simulink model "EV_Battery_Discharge_Regen"  (R2023b)
settings: Solver=FixedStepDiscrete  StartTime=0.0  StopTime=1800  FixedStep=.05  RelTol=1e-3
model workspace (MAT data in the model file):
  observer_parameters = [379.525650451 0.0229436828398 29.3915870716 0.534292035398 0.030625 118.171428571 114.285714286 0.1 10]
undefined symbols (not defined in the file or in its folder): Ion, Lithium
libraries: spsControlledCurrentSourceLib x2, spsCurrentMeasurementLib x1, spsGroundLib x1, spsVoltageMeasurementLib x1, spsBatteryLib x1, sps_lib x1
settings Model: Creator=smitp  LastModifiedBy=smitp

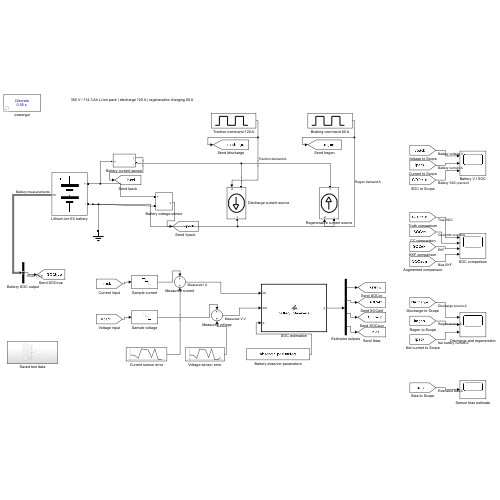
[thumbnail: Simulink's stored preview of the top-level diagram]
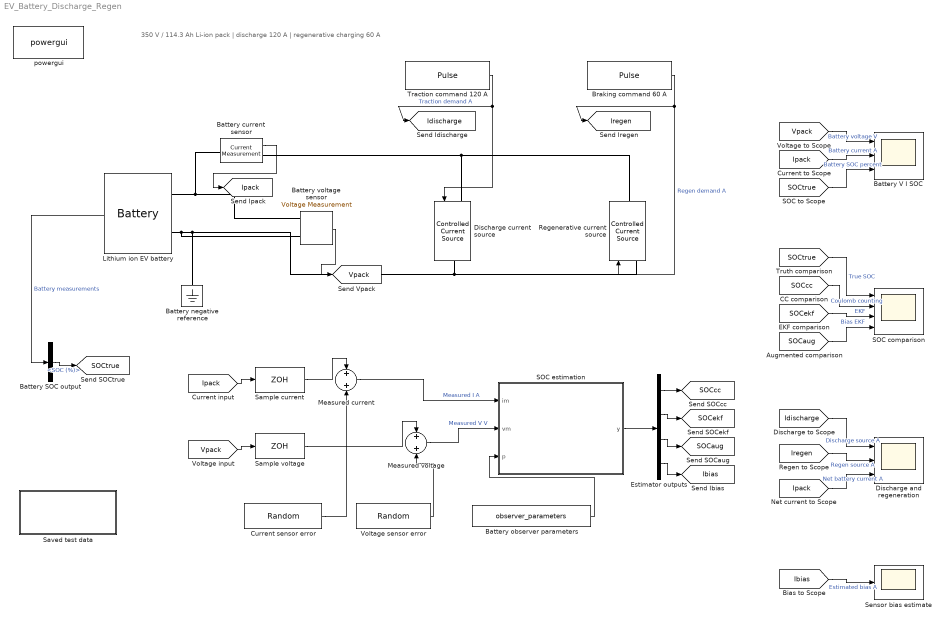
== system EV_Battery_Discharge_Regen ==
  note: 350 V / 114.3 Ah Li-ion pack | discharge 120 A | regenerative charging 60 A
  Battery SOC output : BusSelector  Description=Selects built-in SOC (%) from the Battery measurement bus. It is comparison truth and is never an estimator input.  OutputSignals=SOC (%)
  Battery V I SOC : Scope  NumInputPorts=3
      settings: Description=Primary Scope: voltage, signed battery current and built-in SOC on separate axes.
  Battery current sensor : spsCurrentMeasurementLib/Current Measurement  Description=Measures total battery current. Positive means discharge; negative means charging.  PhasorSimulation=off  OutputType=Complex  PSBequivalent=0
  Battery negative reference : spsGroundLib/Ground  Description=Defines the negative electrical reference node.  LConnTagsString=a
  Battery observer parameters : Constant  Description=Stores E0,K,A,B,R,Qinternal,Qrated,kc,tau extracted from this Battery mask. Contains no true SOC.  Value=observer_parameters
  Battery voltage sensor : spsVoltageMeasurementLib/Voltage Measurement  Description=Connected across the battery terminals to measure pack voltage without drawing current.  PhasorSimulation=off  OutputType=Complex  PSBequivalent=0
  Braking command 60 A : DiscretePulseGenerator  Description=Regeneration is ON from 420 to 540 s in each 600 s cycle, separate from traction.  PulseType=Time based  Amplitude=60  Period=600  PulseWidth=20  PhaseDelay=420
  Current sensor error : RandomNumber  Description=Adds a known +1.2 A offset and 0.25 A standard deviation noise to test current-sensor error.  Mean=1.2  Variance=.25^2  Seed=23  SampleTime=1
  Discharge and regeneration : Scope  NumInputPorts=3
      settings: Description=Shows two nonnegative branch source commands and measured signed net battery current. Ideal-source branch currents equal their commands.
  Discharge current source : spsControlledCurrentSourceLib/Controlled Current Source  Description=Physical current-source load: draws 120 A from HV+ to HV- while traction pulse is high.  Initialize=on  Source_Type=DC  Amplitude=0  Phase=0  Frequency=0  Measurements=None
  Estimator outputs : Demux  Description=Separates the four observer outputs: CC percent, EKF percent, bias-EKF percent, estimated bias A.
  Lithium ion EV battery : spsBatteryLib/Battery  Description=Actual SPS Battery block with internal charge state and nonlinear charge/discharge voltage. This single block represents an EV pack, not a single 350 V cell.  BatType=Lithium-Ion  ShowTempParam=off  ThermalPreset=no  ShowAgeParam=off  NomV=350  NomQ=114.2857142857  SOC=80  Batt_Tr=30  PresetModel=on  MaxQ=114.2857  MinV=262.5  FullV=407.3955  Dis_rate=49.6894  R=0.030625  Normal_OP=103.354  expZone="[378.135      5.614907]"  current=[60 120 180]  Units=Time  Tci=20  NomT=20  T2=-30  MaxQ2=4.8  FullV2=7.1  Normal_OP2=5.655  expZone2="[6.58           1]"  Rca=0.6  ti=2000  Dp=0  Neq0=0  Tsim=1e6  Ta1=25  Qeol=5.4*0.9  Reol=0.013333*1.2  Char_age=[2.3478, 3]  Dis_age=[2.3478, 10]  N1=1500  N2=10500  N3=1000  N4=1400  Ta2=45  N5=950
  Measured current : Sum  Description=Combines true measured current with the current-sensor error.
  Measured voltage : Sum  Description=Combines true terminal voltage with voltage-sensor noise.
  Regenerative current source : spsControlledCurrentSourceLib/Controlled Current Source  Description=Separate physical current source connected in the opposite direction: injects 60 A into the battery positive terminal during braking.  Initialize=on  Source_Type=DC  Amplitude=0  Phase=0  Frequency=0  Measurements=None
  SOC comparison : Scope  NumInputPorts=4
      settings: Description=Shows true SOC, Coulomb counting, EKF and bias-EKF together in percent.
  SOC estimation : MATLAB Function  Description=Online CC, EKF and augmented EKF. States are SOC and filtered current; the augmented filter adds current bias. All priors start at 60 percent.  TreatAsAtomicUnit=on
  Sample current : ZeroOrderHold  Description=Samples measured current once per second for the observer.
  Sample voltage : ZeroOrderHold  Description=Samples terminal voltage at the same 1-second observer rate.
  Saved test data : Subsystem  Description=Records the same Scope signals at 1 s for automated checks and the results table.
  Sensor bias estimate : Scope
      settings: Description=Displays the augmented EKF current-offset estimate. The injected offset is 1.2 A.
  Traction command 120 A : DiscretePulseGenerator  Description=Traction is ON from 60 to 360 s in each 600 s cycle.  PulseType=Time based  Amplitude=120  Period=600  PulseWidth=50  PhaseDelay=60
  Voltage sensor error : RandomNumber  Description=Adds 0.15 V standard deviation pack-voltage noise, with a repeatable independent seed.  Variance=.15^2  Seed=47  SampleTime=1
  powergui : sps_lib/powergui  Description=Solves the connected SPS electrical network. Discrete 50 ms is suitable for this battery current-profile test, not PWM switching.  Priority=1  SimulationMode=Discrete  SampleTime=.05  frequency=60  Iterations=50  frequencyindice=0  Pbase=100e6  ErrMax=1e-4  UnitsV=kV  UnitsW=MW  buscounter=0  FunctionMessages=off  echomessages=off  EnableUseOfTLC=off  CurrentSourceSwitches=off  DisableSnubberDevices=off  DisableRonSwitches=off  DisableVfSwitches=off  DisplayEquations=off  AutomaticDiscreteSolvers=off  SolverType=Tustin/Backward Euler (TBE)  Interpol=off  ExternalGateDelay=off  methode=off  Ts=100  x0status=blocks  SPID=on  SwTol=0  HookPort=off  NonlinearTolerance=1e-4  nMaxIteration=100  ContinueOnMaxIteration=off  RestoreLinks=warning  ResistiveCurrentMeasurement=off  Frange=[0:2:500]  Ylog=off  Xlog=on  ShowGrid=off  save=off  variable=ZData  structure=0  ZoomFFT=off  StartTime=0.0  cycles=1  DisplayStyle=1  fundamental=60  FreqAxis=off  MaxFrequency=1000  frequencyindicesteady=1  RmsSteady=1  display=off
  tag scope: Ibias=global, Idischarge=global, Ipack=global, Iregen=global, SOCaug=global, SOCcc=global, SOCekf=global, SOCtrue=global, Vpack=global
  wires:
  Traction command 120 A/1 -> Discharge current source/1, [Idischarge]  "Traction demand A"
  Braking command 60 A/1 -> Regenerative current source/1, [Iregen]  "Regen demand A"
  Lithium ion EV battery/1 -> Battery SOC output/1  "Battery measurements"
  Battery current sensor/1 -> [Ipack]
  Battery voltage sensor/1 -> [Vpack]
  Battery SOC output/1 -> [SOCtrue]  "<SOC (%)>"
  [Ipack] -> Sample current/1
  [Vpack] -> Sample voltage/1
  Sample current/1 -> Measured current/1
  Current sensor error/1 -> Measured current/2
  Sample voltage/1 -> Measured voltage/1
  Voltage sensor error/1 -> Measured voltage/2
  Measured current/1 -> SOC estimation/1(im)  "Measured I A"
  Measured voltage/1 -> SOC estimation/2(vm)  "Measured V V"
  Battery observer parameters/1 -> SOC estimation/3(p)
  SOC estimation/1(y) -> Estimator outputs/1
  Estimator outputs/1 -> [SOCcc]
  Estimator outputs/2 -> [SOCekf]
  Estimator outputs/3 -> [SOCaug]
  Estimator outputs/4 -> [Ibias]
  [Vpack] -> Battery V I SOC/1  "Battery voltage V"
  [Ipack] -> Battery V I SOC/2  "Battery current A"
  [SOCtrue] -> Battery V I SOC/3  "Battery SOC percent"
  [SOCtrue] -> SOC comparison/1  "True SOC"
  [SOCcc] -> SOC comparison/2  "Coulomb counting"
  [SOCekf] -> SOC comparison/3  "EKF"
  [SOCaug] -> SOC comparison/4  "Bias EKF"
  [Idischarge] -> Discharge and regeneration/1  "Discharge source A"
  [Iregen] -> Discharge and regeneration/2  "Regen source A"
  [Ipack] -> Discharge and regeneration/3  "Net battery current A"
  [Ibias] -> Sensor bias estimate/1  "Estimated bias A"
  connections:
  Battery current sensor/LConn1 -- Lithium ion EV battery/LConn1 -- Battery voltage sensor/LConn1
  Discharge current source/LConn1 -- Battery current sensor/RConn1 -- Regenerative current source/RConn1
  Discharge current source/RConn1 -- Lithium ion EV battery/LConn2 -- Battery voltage sensor/LConn2 -- Battery negative reference/LConn1 -- Regenerative current source/LConn1

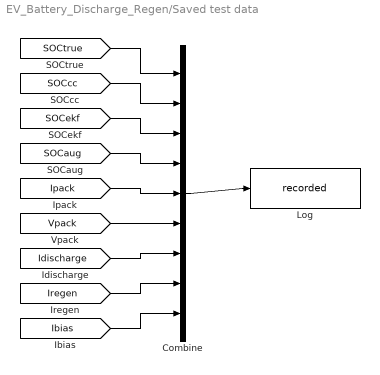
== system EV_Battery_Discharge_Regen/Saved test data ==
  Combine : Mux  Description=Combines nine scalar channels in the documented order.  Inputs=9
  Log : ToWorkspace  VariableName=recorded  SaveFormat=Timeseries  SampleTime=1
      settings: Description=Saves all nine channels as a timeseries named recorded, at 1 s; Scopes remain the primary output.
  wires:
  [SOCtrue] -> Combine/1
  [SOCcc] -> Combine/2
  [SOCekf] -> Combine/3
  [SOCaug] -> Combine/4
  [Ipack] -> Combine/5
  [Vpack] -> Combine/6
  [Idischarge] -> Combine/7
  [Iregen] -> Combine/8
  [Ibias] -> Combine/9
  Combine/1 -> Log/1

== matlab function EV_Battery_Discharge_Regen/SOC estimation ==
  data: im input; y output; vm input; p input
function y=battery_observers(im,vm,p)
% p=[E0 K A B R Qinternal Qrated kc tau]. Current positive on discharge.
% Outputs: CC %, EKF %, augmented EKF %, estimated current offset A.
persistent cc x P xb Pb previousI
if isempty(cc)
 cc=.6; x=[.6;0]; P=diag([.15^2 25]);
 xb=[.6;0;0]; Pb=diag([.15^2 25 1]); previousI=im;
else
 a=exp(-1/p(9)); q=3600*p(7);
 cc=min(1,max(0,cc-previousI/q));
 F=[1 0;0 a]; G=[-1/q;1-a];
 x=F*x+G*previousI; P=F*P*F'+diag([1e-8 .1]);
 Fb=[1 0 1/q;0 a -(1-a);0 0 1];
 xb=Fb*xb+[G;0]*previousI; Pb=Fb*Pb*Fb'+diag([1e-8 .1 1e-5]);
end
x(1)=min(.99,max(.05,x(1))); xb(1)=min(.99,max(.05,xb(1)));
v=terminal(x(1),x(2),im,p); H=zeros(1,2);
H(1)=(terminal(x(1)+1e-5,x(2),im,p)-terminal(x(1)-1e-5,x(2),im,p))/2e-5;
H(2)=(terminal(x(1),x(2)+1e-3,im,p)-terminal(x(1),x(2)-1e-3,im,p))/2e-3;
R=.2^2; K=P*H'/(H*P*H'+R); x=x+K*(vm-v); J=eye(2)-K*H; P=J*P*J'+K*R*K';
vb=terminal(xb(1),xb(2),im-xb(3),p); Hb=zeros(1,3);
Hb(1)=(terminal(xb(1)+1e-5,xb(2),im-xb(3),p)-terminal(xb(1)-1e-5,xb(2),im-xb(3),p))/2e-5;
Hb(2)=(terminal(xb(1),xb(2)+1e-3,im-xb(3),p)-terminal(xb(1),xb(2)-1e-3,im-xb(3),p))/2e-3;
Hb(3)=p(5); Kb=Pb*Hb'/(Hb*Pb*Hb'+R); xb=xb+Kb*(vm-vb); Jb=eye(3)-Kb*Hb; Pb=Jb*Pb*Jb'+Kb*R*Kb';
x(1)=min(1,max(0,x(1))); xb(1)=min(1,max(0,xb(1))); xb(3)=min(5,max(-5,xb(3)));
previousI=im; y=[100*cc;100*x(1);100*xb(1);xb(3)];
end
function v=terminal(z,ifilt,i,p)
it=(1-z)*p(7); Q=p(6);
if ifilt>=0, den=Q-it; else, den=it+Q*p(8); end
v=p(1)-p(2)*Q/(Q-it)*it+p(3)*exp(-p(4)*it)-p(2)*Q/den*ifilt-p(5)*i;
end
